simulink model "simulink_model"  (R2021a)
settings: Solver=ode23tb  StartTime=0.0  StopTime=0.1  MaxStep=0.2e-6  RelTol=1e-3
libraries: spsSeriesRLCBranchLib x4, spsDiodeLib x2, spsVoltageMeasurementLib x2, simulink_extras x1, spsDCVoltageSourceLib x1, spsMosfetLib x1, spsMultimeterLib x1, spspowerguiLib x1
settings Model: Creator=User  LastModifiedBy=User
settings SolverCC: SolverResetMethod=Robust

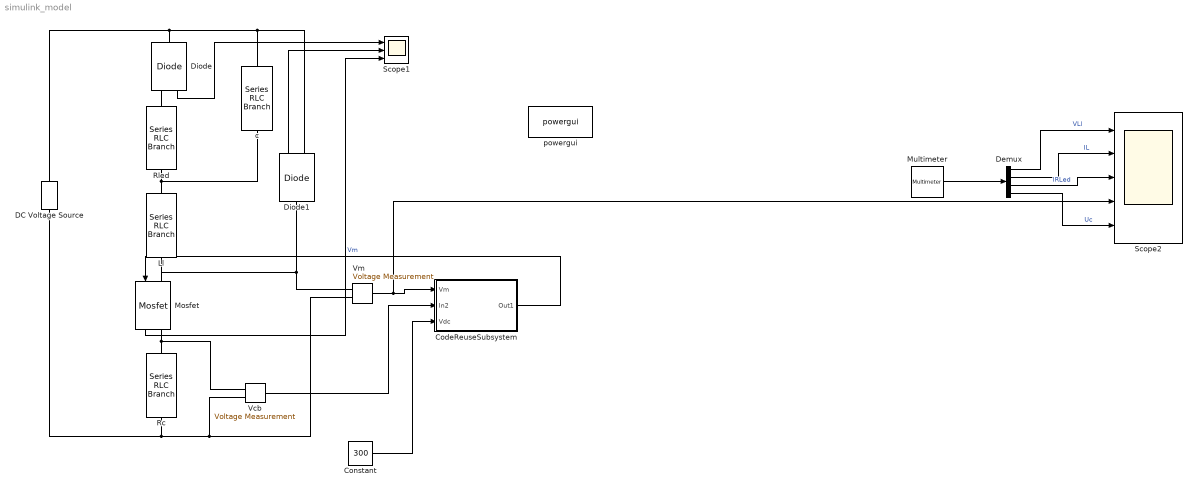
== system simulink_model ==
  CodeReuseSubsystem : Subsystem  TreatAsAtomicUnit=on
      settings: RTWFcnNameOpts=Use subsystem name  RTWFileNameOpts=Use function name
  Constant : Constant  Value=300
  DC Voltage Source : spsDCVoltageSourceLib/DC Voltage Source  Amplitude=300  Measurements=None
  Demux : Demux
  Diode : spsDiodeLib/Diode  Ron=77.7  Lon=0  Vf=85  IC=0  UseSnubber=0  Rs=inf  Cs=250e-9  Measurements=on
  Diode1 : spsDiodeLib/Diode  Ron=0.001  Lon=0  Vf=0.8  IC=0  UseSnubber=0  Rs=inf  Cs=250e-9  Measurements=on
  Ll : spsSeriesRLCBranchLib/Series RLC Branch  LConnTagsString=__new0  RConnTagsString=__new0  BranchType=RL  Resistance=1  Inductance=0.0045  SetiL0=off  InitialCurrent=0  Capacitance=1e-6  Setx0=off  InitialVoltage=0  Measurements=Branch voltage and current
  Mosfet : spsMosfetLib/Mosfet  Ron=0.1  Lon=0  Rd=0.01  Vfd=0  IC=0  Rs=1e5  Cs=inf  Measurements=on
  Multimeter : spsMultimeterLib/Multimeter  PhasorSimulation=off  OutputType=Complex  sel=[1 3 4 2]  L=4  Gain=[1 1 1 1]  yselected={'Ub: Ll','Ib: Ll','Ib: Rled','Ub: c'};  PSBOutputType=1  PSBequivalent=0  AxesSetting=[0,0.1,-100,100]  Display=0  SavedBlockNames=-11
  Rc : spsSeriesRLCBranchLib/Series RLC Branch  LConnTagsString=__new0  RConnTagsString=__new0  BranchType=R  Resistance=2  Inductance=1e-3  SetiL0=off  InitialCurrent=0  Capacitance=1e-6  Setx0=off  InitialVoltage=0  Measurements=None
  Rled : spsSeriesRLCBranchLib/Series RLC Branch  LConnTagsString=__new0  RConnTagsString=__new0  BranchType=R  Resistance=0.1  Inductance=1e-3  SetiL0=off  InitialCurrent=0  Capacitance=1e-6  Setx0=off  InitialVoltage=0  Measurements=Branch current
  Scope1 : Scope  NumInputPorts=3
  Scope2 : Scope  NumInputPorts=5
  Vcb : spsVoltageMeasurementLib/Voltage Measurement  PhasorSimulation=off  OutputType=Complex  PSBequivalent=0
  Vm : spsVoltageMeasurementLib/Voltage Measurement  PhasorSimulation=off  OutputType=Complex  PSBequivalent=0
  c : spsSeriesRLCBranchLib/Series RLC Branch  LConnTagsString=__new0  RConnTagsString=__new0  BranchType=RC  Resistance=1.38  Inductance=1e-3  SetiL0=off  InitialCurrent=0  Capacitance=0.000004  Setx0=off  InitialVoltage=0  Measurements=Branch voltage
  powergui : spspowerguiLib/powergui  Priority=1  SimulationMode=Continuous  SampleTime=50e-6  frequency=60  Iterations=50  frequencyindice=0  Pbase=100e6  ErrMax=1e-4  UnitsV=kV  UnitsW=MW  buscounter=0  FunctionMessages=off  echomessages=off  EnableUseOfTLC=off  CurrentSourceSwitches=off  DisableSnubberDevices=off  DisableRonSwitches=off  DisableVfSwitches=off  DisplayEquations=off  AutomaticDiscreteSolvers=off  SolverType=Tustin/Backward Euler (TBE)  Interpol=off  ExternalGateDelay=off  methode=off  Ts=100  x0status=blocks  SPID=on  SwTol=0  HookPort=off  NonlinearTolerance=1e-4  nMaxIteration=100  ContinueOnMaxIteration=off  RestoreLinks=warning  ResistiveCurrentMeasurement=off  Frange=[0:2:500]  Ylog=off  Xlog=on  ShowGrid=off  save=off  variable=ZData  structure=0  ZoomFFT=off  StartTime=0.0  cycles=1  DisplayStyle=1  fundamental=60  FreqAxis=off  MaxFrequency=1000  frequencyindicesteady=1  RmsSteady=1  display=off
  wires:
  Vm/1 -> Scope2/4, CodeReuseSubsystem/1(Vm)
  Vcb/1 -> CodeReuseSubsystem/2(In2)
  Constant/1 -> CodeReuseSubsystem/3(Vdc)
  CodeReuseSubsystem/1(Out1) -> Mosfet/1  "Vm"
  Mosfet/1 -> Scope1/3
  Diode/1 -> Scope1/1
  Diode1/1 -> Scope1/2
  Multimeter/1 -> Demux/1
  Demux/3 -> Scope2/3  "IRLed"
  Demux/2 -> Scope2/2  "IL"
  Demux/1 -> Scope2/1  "VLl"
  Demux/4 -> Scope2/5  "Uc"
  connections:
  Rc/LConn1 -- Vcb/LConn1 -- Mosfet/RConn1
  DC Voltage Source/RConn1 -- Diode/LConn1 -- Diode1/RConn1 -- c/LConn1
  Diode1/LConn1 -- Mosfet/LConn1 -- Ll/RConn1 -- Vm/LConn1
  Rc/RConn1 -- DC Voltage Source/LConn1 -- Vcb/LConn2 -- Vm/LConn2
  Rled/LConn1 -- Diode/RConn1
  c/RConn1 -- Ll/LConn1 -- Rled/RConn1

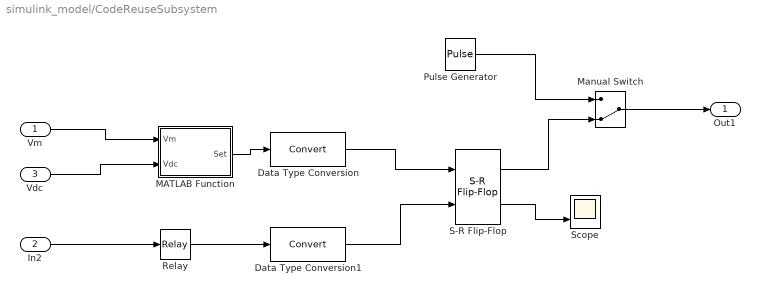
== system simulink_model/CodeReuseSubsystem ==
  Vm : Inport
  In2 : Inport  Port=2
  Vdc : Inport  Port=3
  Data Type Conversion : DataTypeConversion
  Data Type Conversion1 : DataTypeConversion
  MATLAB Function : MATLAB Function  TreatAsAtomicUnit=on
  Manual Switch : ManualSwitch  CurrentSetting=0
  Pulse Generator : DiscretePulseGenerator  PulseType=Time based  Amplitude=5  Period=1/50000  PulseWidth=45
  Relay : Relay  OnSwitchValue=0.4  OffSwitchValue=0.39
  S-R Flip-Flop : simulink_extras/Flip Flops/S-R Flip-Flop  initial_condition=0
  Scope : Scope  NumInputPorts=2
  Out1 : Outport
  wires:
  Vm/1 -> MATLAB Function/1(Vm)
  Vdc/1 -> MATLAB Function/2(Vdc)
  In2/1 -> Relay/1
  Relay/1 -> Data Type Conversion1/1
  MATLAB Function/1(Set) -> Data Type Conversion/1
  Data Type Conversion/1 -> S-R Flip-Flop/1
  Data Type Conversion1/1 -> S-R Flip-Flop/2
  Manual Switch/1 -> Out1/1
  S-R Flip-Flop/2 -> Scope/2
  Pulse Generator/1 -> Manual Switch/1
  S-R Flip-Flop/1 -> Manual Switch/2

== matlab function simulink_model/CodeReuseSubsystem/MATLAB Function ==
  data: Vm input; Set output; Vdc input
function Set = fcn(Vm, Vdc)

    if ( Vm <( Vdc-40) && Vm>20 )
        Set=1;
        
    else Set=0;
        
    end;

end
